simulink library "Contact_Forces_Lib"  (R2024a)
settings: Solver=ode45  StartTime=0.0  StopTime=10.0  RelTol=1e-3  EnableMultiTasking=on
undefined symbols (not defined in the file or in its folder): b_contact, custom_param_1, custom_param_2, Extr_Data_Ring, k_contact, l_cone, length_cylinder, length_tube, mu_kinetic, mu_static, pen_exponent, pen_full_damp_F, rad_s_cone, radius_cylinder, radius_tube, v_thr, X, Y, Z
libraries: nesl_utility x197, sm_lib x115, $bdroot x72, simulink x20, fl_lib x4
(part 10 of 12)

== system Contact_Forces_Lib/3D/Sphere to Tube Force/Forces/Sum ==
  FnxSphF : Inport
  FnySphF : Inport  Port=2
  FnzSphF : Inport  Port=3
  FnxTubB : Inport  Port=4
  FnyTubB : Inport  Port=5
  TnxTubB : Inport  Port=6
  TnyTubB : Inport  Port=7
  FfxSphF : Inport  Port=8
  FfySphF : Inport  Port=9
  FfzSphF : Inport  Port=10
  FfxTubB : Inport  Port=11
  FfyTubB : Inport  Port=12
  FfzTubB : Inport  Port=13
  TzSphF : Inport  Port=14
  TTubB : Inport  Port=15
  Constant : Constant  Value=0
  Mux : Mux  Inputs=3
  Sum{1..6} (6 alike) : Sum
  FxF : Outport  VectorParamsAs1DForOutWhenUnconnected=off
  FyF : Outport  Port=2  VectorParamsAs1DForOutWhenUnconnected=off
  FzF : Outport  Port=3  VectorParamsAs1DForOutWhenUnconnected=off
  TzF : Outport  Port=4  VectorParamsAs1DForOutWhenUnconnected=off
  FxB : Outport  Port=5  VectorParamsAs1DForOutWhenUnconnected=off
  FyB : Outport  Port=6  VectorParamsAs1DForOutWhenUnconnected=off
  FzB : Outport  Port=7  VectorParamsAs1DForOutWhenUnconnected=off
  TB : Outport  Port=8  VectorParamsAs1DForOutWhenUnconnected=off
  wires:
  Sum6/1 -> TB/1
  FfzTubB/1 -> FzB/1
  FfzSphF/1 -> Sum1/2
  FnzSphF/1 -> Sum1/1
  Sum1/1 -> FzF/1
  FnxSphF/1 -> Sum4/1
  FnySphF/1 -> Sum2/1
  FnxTubB/1 -> Sum3/1
  FnyTubB/1 -> Sum5/1
  Sum4/1 -> FxF/1
  Sum2/1 -> FyF/1
  Sum3/1 -> FxB/1
  Sum5/1 -> FyB/1
  FfxSphF/1 -> Sum4/2
  FfySphF/1 -> Sum2/2
  FfxTubB/1 -> Sum3/2
  FfyTubB/1 -> Sum5/2
  TzSphF/1 -> TzF/1
  TTubB/1 -> Sum6/1
  Mux/1 -> Sum6/2
  TnxTubB/1 -> Mux/1
  TnyTubB/1 -> Mux/2
  Constant/1 -> Mux/3

== system Contact_Forces_Lib/3D/Sphere to Tube Force/Sensing/rad_azm_cal ==
  X : Inport
  Y : Inport  Port=2
  Xdot : Inport  Port=3
  Ydot : Inport  Port=4
  Demux : Demux
  If centers are not colocated : If  IfExpression=(u1 > 0)
  Math Function : Math  Operator=square  SignedPower=on
  Math Function1 : Math  Operator=square  SignedPower=on
  Merge : Merge  InitialOutput=0  InputPortOffsets=0
  Sum : Sum  Inputs=|++
  rad_0 : Subsystem
  rad_azm_cal : Subsystem
  rad : Outport  VectorParamsAs1DForOutWhenUnconnected=off
  azm : Outport  Port=2  VectorParamsAs1DForOutWhenUnconnected=off
  radv : Outport  Port=3  VectorParamsAs1DForOutWhenUnconnected=off
  azmv : Outport  Port=4  VectorParamsAs1DForOutWhenUnconnected=off
  wires:
  Sum/1 -> If centers are not colocated/1
  Math Function/1 -> Sum/1
  Math Function1/1 -> Sum/2
  rad_azm_cal/1(F) -> Merge/2
  Y/1 -> rad_azm_cal/2(Y), Math Function1/1
  Ydot/1 -> rad_azm_cal/4(Ydot)
  X/1 -> rad_azm_cal/1(X), Math Function/1
  Xdot/1 -> rad_azm_cal/3(Xdot)
  Demux/3 -> radv/1
  Demux/1 -> rad/1
  Demux/4 -> azmv/1
  rad_0/1(F) -> Merge/1
  Demux/2 -> azm/1
  If centers are not colocated/2 -> rad_0/Action
  If centers are not colocated/1 -> rad_azm_cal/Action
  Merge/1 -> Demux/1

== system Contact_Forces_Lib/3D/Sphere to Tube Force Enabled/Check Active/Check Active Range ==
  azm : Inport
  " Upper Bound" : simulink/Logic and Bit Operations/Compare To Constant  relop=<=  const=active_angle(2)*pi/180  OutDataTypeStr=boolean  ZeroCross=off
  Logical Operator : Logic  AllPortsSameDT=off  OutDataTypeStr=boolean
  Lower Bound : simulink/Logic and Bit Operations/Compare To Constant  relop=>=  const=active_angle(1)*pi/180  OutDataTypeStr=boolean  ZeroCross=off
  En : Outport  VectorParamsAs1DForOutWhenUnconnected=off
  wires:
  Logical Operator/1 -> En/1
  Lower Bound/1 -> Logical Operator/2
  " Upper Bound"/1 -> Logical Operator/1
  azm/1 -> Lower Bound/1, " Upper Bound"/1

== system Contact_Forces_Lib/3D/Sphere to Tube Force Enabled/Check Active/In Tube ==
  z : Inport
  Abs1 : Abs  ZeroCross=off  SaturateOnIntegerOverflow=off
  Activation limit for contact force : Constant  Value=l_tube/2
  Sum : Sum  Inputs=+-
  En : Outport  VectorParamsAs1DForOutWhenUnconnected=off
  wires:
  Sum/1 -> En/1
  Activation limit for contact force/1 -> Sum/1
  z/1 -> Abs1/1
  Abs1/1 -> Sum/2

== system Contact_Forces_Lib/3D/Sphere to Tube Force Enabled/Forces/Calculate Penetration ==
  note: Calculates CirF frame to midpoint of ring wall.
      | Absolute value makes it valid for inside or outside contact.
      | Noting the sign allows us to apply the force correctly
  rad : Inport
  vrad : Inport  Port=2
  Abs : Abs  ZeroCross=off  SaturateOnIntegerOverflow=off
  Constant : Constant  Value=radius_sphere+d_tube/2
  Dead Zone : DeadZone  LowerValue=-inf  UpperValue=0
  Product : Product
  Sign : Signum  ZeroCross=off
  Sum : Sum  Inputs=+-
  Sum1 : Sum  Inputs=+-
  radius ring : Constant  Value=radius_tube
  sign : Outport  VectorParamsAs1DForOutWhenUnconnected=off
  Pen : Outport  Port=2  VectorParamsAs1DForOutWhenUnconnected=off
  Pen Vel : Outport  Port=3  VectorParamsAs1DForOutWhenUnconnected=off
  wires:
  Dead Zone/1 -> Pen/1
  Constant/1 -> Sum/1
  Sum/1 -> Dead Zone/1
  vrad/1 -> Product/2
  Product/1 -> Pen Vel/1
  Sign/1 -> sign/1, Product/1
  Abs/1 -> Sum/2
  rad/1 -> Sum1/2
  Sum1/1 -> Abs/1, Sign/1
  radius ring/1 -> Sum1/1

== system Contact_Forces_Lib/3D/Sphere to Tube Force Enabled/Forces/Ff ==
  note: Sign of Fn indicates if sphere is inside or outside tube
  Fn : Inport
  z : Inport  Port=2
  R : Inport  Port=3
  azm : Inport  Port=4
  vazm : Inport  Port=5
  wzf : Inport  Port=6
  Pen : Inport  Port=7
  rad : Inport  Port=8
  vzf : Inport  Port=9
  wxf : Inport  Port=10
  wyf : Inport  Port=11
  Friction Law : $bdroot/Friction Law  SystemSampleTime=-1  LabelModeActiveChoice=Stick_Slip_C  VariantActivationTime=update diagram  AllowFlexibleInterface=on  Latency=0  AutoFrameSizeCalculation=off
  Relative vel at CP : Subsystem
  Resolve Ff : Subsystem
  Sign : Signum  ZeroCross=off
  FxSphF : Outport  VectorParamsAs1DForOutWhenUnconnected=off
  FySohF : Outport  Port=2  VectorParamsAs1DForOutWhenUnconnected=off
  FzSphF : Outport  Port=3  VectorParamsAs1DForOutWhenUnconnected=off
  FxTubB : Outport  Port=4  VectorParamsAs1DForOutWhenUnconnected=off
  FyTubB : Outport  Port=5  VectorParamsAs1DForOutWhenUnconnected=off
  FzTubB : Outport  Port=6  VectorParamsAs1DForOutWhenUnconnected=off
  TSphF : Outport  Port=7  VectorParamsAs1DForOutWhenUnconnected=off
  TTubB : Outport  Port=8  VectorParamsAs1DForOutWhenUnconnected=off
  Ff : Outport  Port=9  VectorParamsAs1DForOutWhenUnconnected=off
  wires:
  Sign/1 -> Resolve Ff/1(InOut)  "InOut"
  z/1 -> Resolve Ff/6(z)
  Relative vel at CP/1(vRelAbs) -> Friction Law/2  "vRelAbs"
  Relative vel at CP/2(rSphtoCP) -> Resolve Ff/3(rSphtoCP)
  Relative vel at CP/3(rCyltoCP) -> Resolve Ff/4(rCyltoCP)
  azm/1 -> Relative vel at CP/9(azm), Resolve Ff/8(azm)
  wyf/1 -> Relative vel at CP/8(wyf)
  wxf/1 -> Relative vel at CP/7(wxf)
  Resolve Ff/8(TTubB) -> TTubB/1
  Resolve Ff/4(TSphF) -> TSphF/1
  Resolve Ff/6(FyTubB) -> FyTubB/1
  Resolve Ff/5(FxSphB) -> FxTubB/1
  Resolve Ff/2(FySphF) -> FySohF/1
  Resolve Ff/1(FxSphF) -> FxSphF/1
  Friction Law/1 -> Resolve Ff/2(Ff), Ff/1  "Ff Abs"
  wzf/1 -> Relative vel at CP/5(wzf)
  vazm/1 -> Relative vel at CP/4(vazm)
  rad/1 -> Relative vel at CP/2(rad)
  Fn/1 -> Sign/1, Friction Law/1, Relative vel at CP/1(Fn)  "Fn"
  Pen/1 -> Relative vel at CP/3(Pen)
  R/1 -> Resolve Ff/7(R)
  vzf/1 -> Relative vel at CP/6(vzf)
  Relative vel at CP/4(alpha) -> Resolve Ff/5(alpha)
  Resolve Ff/3(FzSphF) -> FzSphF/1
  Resolve Ff/7(FzTubB) -> FzTubB/1

== system Contact_Forces_Lib/3D/Sphere to Tube Force Enabled/Forces/Fn ==
  note: Resolve Normal Force in
      | Sphere F reference frame
  note: Resolve Normal Force in
      | Tube B reference frame
  Fn : Inport
  z : Inport  Port=2
  R : Inport  Port=3
  azm : Inport  Port=4
  Fn in SphF : Subsystem
  Fn in TubB : Subsystem
  Gain : Gain  Gain=-1
  Product : Product
  Product1 : Product
  FxSphF : Outport  VectorParamsAs1DForOutWhenUnconnected=off
  FySphF : Outport  Port=2  VectorParamsAs1DForOutWhenUnconnected=off
  FZSphF : Outport  Port=3  VectorParamsAs1DForOutWhenUnconnected=off
  FxTubB : Outport  Port=4  VectorParamsAs1DForOutWhenUnconnected=off
  FyTubB : Outport  Port=5  VectorParamsAs1DForOutWhenUnconnected=off
  TxTubB : Outport  Port=6  VectorParamsAs1DForOutWhenUnconnected=off
  TyTubB : Outport  Port=7  VectorParamsAs1DForOutWhenUnconnected=off
  wires:
  Fn in SphF/3(FzSphF) -> FZSphF/1
  Fn in SphF/2(FxSphF) -> FxSphF/1
  R/1 -> Fn in SphF/1(R)
  azm/1 -> Fn in TubB/2(azm)
  Fn/1 -> Fn in TubB/1(Fn)
  Fn in TubB/2(FyTubB) -> Fn in SphF/3(FyTubB), FyTubB/1, Gain/1
  Fn in TubB/1(FxTubB) -> Fn in SphF/2(FxTubB), Product/2, FxTubB/1
  Fn in SphF/1(FySphF) -> FySphF/1
  z/1 -> Product1/1, Product/1
  Gain/1 -> Product1/2
  Product/1 -> TyTubB/1
  Product1/1 -> TxTubB/1

== system Contact_Forces_Lib/3D/Sphere to Tube Force Enabled/Forces/Sum ==
  FnxSphF : Inport
  FnySphF : Inport  Port=2
  FnzSphF : Inport  Port=3
  FnxTubB : Inport  Port=4
  FnyTubB : Inport  Port=5
  TnxTubB : Inport  Port=6
  TnyTubB : Inport  Port=7
  FfxSphF : Inport  Port=8
  FfySphF : Inport  Port=9
  FfzSphF : Inport  Port=10
  FfxTubB : Inport  Port=11
  FfyTubB : Inport  Port=12
  FfzTubB : Inport  Port=13
  TzSphF : Inport  Port=14
  TTubB : Inport  Port=15
  Constant : Constant  Value=0
  Mux : Mux  Inputs=3
  Sum{1..6} (6 alike) : Sum
  FxF : Outport  VectorParamsAs1DForOutWhenUnconnected=off
  FyF : Outport  Port=2  VectorParamsAs1DForOutWhenUnconnected=off
  FzF : Outport  Port=3  VectorParamsAs1DForOutWhenUnconnected=off
  TzF : Outport  Port=4  VectorParamsAs1DForOutWhenUnconnected=off
  FxB : Outport  Port=5  VectorParamsAs1DForOutWhenUnconnected=off
  FyB : Outport  Port=6  VectorParamsAs1DForOutWhenUnconnected=off
  FzB : Outport  Port=7  VectorParamsAs1DForOutWhenUnconnected=off
  TB : Outport  Port=8  VectorParamsAs1DForOutWhenUnconnected=off
  wires:
  Sum6/1 -> TB/1
  FfzTubB/1 -> FzB/1
  FfzSphF/1 -> Sum1/2
  FnzSphF/1 -> Sum1/1
  Sum1/1 -> FzF/1
  FnxSphF/1 -> Sum4/1
  FnySphF/1 -> Sum2/1
  FnxTubB/1 -> Sum3/1
  FnyTubB/1 -> Sum5/1
  Sum4/1 -> FxF/1
  Sum2/1 -> FyF/1
  Sum3/1 -> FxB/1
  Sum5/1 -> FyB/1
  FfxSphF/1 -> Sum4/2
  FfySphF/1 -> Sum2/2
  FfxTubB/1 -> Sum3/2
  FfyTubB/1 -> Sum5/2
  TzSphF/1 -> TzF/1
  TTubB/1 -> Sum6/1
  Mux/1 -> Sum6/2
  TnxTubB/1 -> Mux/1
  TnyTubB/1 -> Mux/2
  Constant/1 -> Mux/3

== system Contact_Forces_Lib/3D/Sphere to Tube Force Enabled/Sensing/In or Out ==
  rad : Inport
  Constant : Constant  Value=radius_tube
  Constant1 : Constant  Value=-d_tube/2
  Constant2 : Constant  Value=radius_tube
  Product : Product
  Product1 : Product
  Sign : Signum  ZeroCross=off
  Subtract : Sum  Inputs=+-
  Sum : Sum
  factor : Outport  VectorParamsAs1DForOutWhenUnconnected=off
  wires:
  Constant/1 -> Subtract/1
  Sign/1 -> Product/1, Product1/1
  Subtract/1 -> Sign/1
  rad/1 -> Subtract/2
  Constant1/1 -> Product/2
  Product/1 -> Sum/1
  Sum/1 -> Product1/2
  Product1/1 -> factor/1
  Constant2/1 -> Sum/2

== system Contact_Forces_Lib/3D/Sphere to Tube Force Enabled/Sensing/rad_azm_cal ==
  X : Inport
  Y : Inport  Port=2
  Xdot : Inport  Port=3
  Ydot : Inport  Port=4
  Demux : Demux
  If centers are not colocated : If  IfExpression=(u1 > 0)
  Math Function : Math  Operator=square  SignedPower=on
  Math Function1 : Math  Operator=square  SignedPower=on
  Merge : Merge  InitialOutput=0  InputPortOffsets=0
  Sum : Sum  Inputs=|++
  rad_0 : Subsystem
  rad_azm_cal : Subsystem
  rad : Outport  VectorParamsAs1DForOutWhenUnconnected=off
  azm : Outport  Port=2  VectorParamsAs1DForOutWhenUnconnected=off
  radv : Outport  Port=3  VectorParamsAs1DForOutWhenUnconnected=off
  azmv : Outport  Port=4  VectorParamsAs1DForOutWhenUnconnected=off
  wires:
  Sum/1 -> If centers are not colocated/1
  Math Function/1 -> Sum/1
  Math Function1/1 -> Sum/2
  rad_azm_cal/1(F) -> Merge/2
  Y/1 -> rad_azm_cal/2(Y), Math Function1/1
  Ydot/1 -> rad_azm_cal/4(Ydot)
  X/1 -> rad_azm_cal/1(X), Math Function/1
  Xdot/1 -> rad_azm_cal/3(Xdot)
  Demux/3 -> radv/1
  Demux/1 -> rad/1
  Demux/4 -> azmv/1
  rad_0/1(F) -> Merge/1
  Demux/2 -> azm/1
  If centers are not colocated/2 -> rad_0/Action
  If centers are not colocated/1 -> rad_azm_cal/Action
  Merge/1 -> Demux/1

== system Contact_Forces_Lib/Friction Utilities/Utilities/Product/FcConst ==
  PS Product : fl_lib/Physical Signals/Functions/PS Product
  PS Terminator : fl_lib/Physical Signals/Sinks/PS Terminator
  Fc : PMIOPort  Side=Right
  v : PMIOPort  Port=2  Side=Right
  connections:
  PS Product/LConn1 -- v/RConn1
  PS Product/LConn2 -- Fc/RConn1
  PS Terminator/LConn1 -- PS Product/RConn1

== system Contact_Forces_Lib/Friction Utilities/Utilities/Product/FcVect ==
  PS Terminator : fl_lib/Physical Signals/Sinks/PS Terminator
  PS Terminator1 : fl_lib/Physical Signals/Sinks/PS Terminator
  Fc : PMIOPort  Side=Right
  v : PMIOPort  Port=2  Side=Right
  connections:
  PS Terminator1/LConn1 -- Fc/RConn1
  PS Terminator/LConn1 -- v/RConn1

== system Contact_Forces_Lib/2D/Circle to Circle Force/Ff/Resolve Ff/Ff in CirB ==
  Ff : Inport
  azm : Inport  Port=2
  Divide1 : Product  Inputs=**
  Divide2 : Product  Inputs=**
  Gain3 : Gain  Gain=-1
  cos : Trigonometry
  deg2rad : Gain  Gain=pi/180
  sin : Trigonometry  Operator=cos
  FxCirB : Outport  VectorParamsAs1DForOutWhenUnconnected=off
  FyCirB : Outport  Port=2  VectorParamsAs1DForOutWhenUnconnected=off
  wires:
  Gain3/1 -> Divide1/2
  Ff/1 -> Divide1/1, Divide2/1
  Divide1/1 -> FxCirB/1
  deg2rad/1 -> cos/1, sin/1
  sin/1 -> Divide2/2
  cos/1 -> Gain3/1
  Divide2/1 -> FyCirB/1  "Fy Cir"
  azm/1 -> deg2rad/1

== system Contact_Forces_Lib/2D/Circle to Circle Force/Ff/Resolve Ff/Ff in CirF ==
  R : Inport
  FxCirB : Inport  Port=2
  FyCirB : Inport  Port=3
  Demux : Demux  Outputs=2
  Divide3 : Product  Inputs=**  Multiplication=Matrix(*)
  Gain1 : Gain  Gain=-1
  Mux1 : Mux  Inputs=2
  FyCirF : Outport  VectorParamsAs1DForOutWhenUnconnected=off
  FxCirF : Outport  Port=2  VectorParamsAs1DForOutWhenUnconnected=off
  wires:
  FxCirB/1 -> Mux1/2
  FyCirB/1 -> Mux1/1
  Demux/2 -> FxCirF/1
  Demux/1 -> FyCirF/1
  Gain1/1 -> Demux/1
  Mux1/1 -> Divide3/2
  Divide3/1 -> Gain1/1
  R/1 -> Divide3/1

== system Contact_Forces_Lib/2D/Circle to Circle Force/Ff/Resolve Ff/Tz ==
  rCirFtoCP : Inport
  rCirBtoCP : Inport  Port=2
  Ff : Inport  Port=3
  Divide4 : Product  Inputs=**
  Divide5 : Product  Inputs=**
  Gain2 : Gain
  TzB : Outport  VectorParamsAs1DForOutWhenUnconnected=off
  TzF : Outport  Port=2  VectorParamsAs1DForOutWhenUnconnected=off
  wires:
  Ff/1 -> Divide4/1, Gain2/1
  Gain2/1 -> Divide5/1
  Divide4/1 -> TzF/1
  rCirFtoCP/1 -> Divide4/2
  Divide5/1 -> TzB/1
  rCirBtoCP/1 -> Divide5/2

== system Contact_Forces_Lib/2D/Circle to Circle Force Enabled/Ff/Resolve Ff/Ff in CirB ==
  Ff : Inport
  azm : Inport  Port=2
  Divide1 : Product  Inputs=**
  Divide2 : Product  Inputs=**
  Gain3 : Gain  Gain=-1
  cos : Trigonometry
  deg2rad : Gain  Gain=pi/180
  sin : Trigonometry  Operator=cos
  FxCirB : Outport  VectorParamsAs1DForOutWhenUnconnected=off
  FyCirB : Outport  Port=2  VectorParamsAs1DForOutWhenUnconnected=off
  wires:
  azm/1 -> deg2rad/1
  Divide2/1 -> FyCirB/1  "Fy Cir"
  cos/1 -> Gain3/1
  sin/1 -> Divide2/2
  deg2rad/1 -> sin/1, cos/1
  Divide1/1 -> FxCirB/1
  Ff/1 -> Divide2/1, Divide1/1
  Gain3/1 -> Divide1/2

== system Contact_Forces_Lib/2D/Circle to Circle Force Enabled/Ff/Resolve Ff/Ff in CirF ==
  R : Inport
  FxCirB : Inport  Port=2
  FyCirB : Inport  Port=3
  Demux : Demux  Outputs=2
  Divide3 : Product  Inputs=**  Multiplication=Matrix(*)
  Gain1 : Gain  Gain=-1
  Mux1 : Mux  Inputs=2
  FyCirF : Outport  VectorParamsAs1DForOutWhenUnconnected=off
  FxCirF : Outport  Port=2  VectorParamsAs1DForOutWhenUnconnected=off
  wires:
  R/1 -> Divide3/1
  Divide3/1 -> Gain1/1
  Mux1/1 -> Divide3/2
  Gain1/1 -> Demux/1
  Demux/1 -> FyCirF/1
  Demux/2 -> FxCirF/1
  FyCirB/1 -> Mux1/1
  FxCirB/1 -> Mux1/2

== system Contact_Forces_Lib/2D/Circle to Circle Force Enabled/Ff/Resolve Ff/Tz ==
  rCirFtoCP : Inport
  rCirBtoCP : Inport  Port=2
  Ff : Inport  Port=3
  Divide4 : Product  Inputs=**
  Divide5 : Product  Inputs=**
  Gain2 : Gain
  TzB : Outport  VectorParamsAs1DForOutWhenUnconnected=off
  TzF : Outport  Port=2  VectorParamsAs1DForOutWhenUnconnected=off
  wires:
  rCirBtoCP/1 -> Divide5/2
  Divide5/1 -> TzB/1
  rCirFtoCP/1 -> Divide4/2
  Divide4/1 -> TzF/1
  Gain2/1 -> Divide5/1
  Ff/1 -> Gain2/1, Divide4/1

== system Contact_Forces_Lib/2D/Circle to Finite Line Force/Forces/Resolve Forces/FnCir ==
  note: Calculate circle Normal Force in circle reference frame
  Unit Vector : Inport
  Fn : Inport  Port=2
  Demux1 : Demux  Outputs=2
  Divide1 : Product  Inputs=**
  FxCir : Outport  VectorParamsAs1DForOutWhenUnconnected=off
  FyCir : Outport  Port=2  VectorParamsAs1DForOutWhenUnconnected=off
  wires:
  Unit Vector/1 -> Divide1/2
  Divide1/1 -> Demux1/1
  Fn/1 -> Divide1/1
  Demux1/2 -> FyCir/1  "Fy Cir"
  Demux1/1 -> FxCir/1  "Fx Cir"

== system Contact_Forces_Lib/2D/Circle to Finite Line Force/Forces/Resolve Forces/FnLin ==
  note: Normal Force is calculated in line reference frame,
      | and acts along x-axis only.
  Fn : Inport
  Constant : Constant  Value=0
  Constant1 : Constant  Value=0
  Sum : Sum
  FxLin : Outport  VectorParamsAs1DForOutWhenUnconnected=off
  FyLin : Outport  Port=2  VectorParamsAs1DForOutWhenUnconnected=off
  wires:
  Constant1/1 -> Sum/1
  Sum/1 -> FxLin/1
  Fn/1 -> Sum/2  "Fx Lin"
  Constant/1 -> FyLin/1  "Fy Lin"

== system Contact_Forces_Lib/2D/Circle to Finite Line Force/Forces/Resolve Forces/Friction ==
  Unit Vector : Inport
  Fn : Inport  Port=2
  X Sep : Inport  Port=3
  vLin : Inport  Port=4
  wz : Inport  Port=5
  Components : Gain  Gain=[1 -1]
  Demux : Demux  Outputs=2
  Friction Law : $bdroot/Friction Law  SystemSampleTime=-1  LabelModeActiveChoice=None  VariantActivationTime=update diagram  AllowFlexibleInterface=on  Latency=0  AutoFrameSizeCalculation=off
  Line Ref h : Gain  Gain=line_depth
  Product1 : Product
  Product2 : Product
  Product3 : Product
  Radius : Gain  Gain=-circle_rad
  Sign : Signum
  Sum : Sum  Inputs=-+
  VCirPt : Subsystem
  FxCir : Outport  VectorParamsAs1DForOutWhenUnconnected=off
  FyCir : Outport  Port=2  VectorParamsAs1DForOutWhenUnconnected=off
  FyLin : Outport  Port=3  VectorParamsAs1DForOutWhenUnconnected=off
  TzLin : Outport  Port=4  VectorParamsAs1DForOutWhenUnconnected=off
  TzCir : Outport  Port=5  VectorParamsAs1DForOutWhenUnconnected=off
  Ff : Outport  Port=6  VectorParamsAs1DForOutWhenUnconnected=off
  wires:
  Sign/1 -> Product3/2, Product1/2
  X Sep/1 -> VCirPt/2(X sep), Sign/1
  Product2/1 -> Demux/1
  Radius/1 -> TzCir/1
  Line Ref h/1 -> TzLin/1
  Fn/1 -> Friction Law/1
  Sum/1 -> Friction Law/2
  Unit Vector/1 -> Components/1
  wz/1 -> VCirPt/1(wz)
  Demux/2 -> FxCir/1  "FxCir"
  VCirPt/1(vCir) -> Sum/2
  vLin/1 -> Sum/1
  Demux/1 -> FyCir/1  "FyCir"
  Friction Law/1 -> Product1/1, Radius/1, Ff/1, Product2/2, Line Ref h/1  "Ff"
  Product1/1 -> FyLin/1
  Components/1 -> Product3/1
  Product3/1 -> Product2/1

== system Contact_Forces_Lib/2D/Circle to Finite Line Force Enabled/Forces/Resolve Forces/FnCir ==
  note: Calculate circle Normal Force in circle reference frame
  Unit Vector : Inport
  Fn : Inport  Port=2
  Demux1 : Demux  Outputs=2
  Divide1 : Product  Inputs=**
  FxCir : Outport  VectorParamsAs1DForOutWhenUnconnected=off
  FyCir : Outport  Port=2  VectorParamsAs1DForOutWhenUnconnected=off
  wires:
  Demux1/1 -> FxCir/1  "Fx Cir"
  Demux1/2 -> FyCir/1  "Fy Cir"
  Fn/1 -> Divide1/1
  Divide1/1 -> Demux1/1
  Unit Vector/1 -> Divide1/2

== system Contact_Forces_Lib/2D/Circle to Finite Line Force Enabled/Forces/Resolve Forces/FnLin ==
  note: Normal Force is calculated in line reference frame,
      | and acts along x-axis only.
  Fn : Inport
  Constant : Constant  Value=0
  Constant1 : Constant  Value=0
  Sum : Sum
  FxLin : Outport  VectorParamsAs1DForOutWhenUnconnected=off
  FyLin : Outport  Port=2  VectorParamsAs1DForOutWhenUnconnected=off
  wires:
  Constant/1 -> FyLin/1  "Fy Lin"
  Fn/1 -> Sum/2  "Fx Lin"
  Sum/1 -> FxLin/1
  Constant1/1 -> Sum/1

== system Contact_Forces_Lib/2D/Circle to Finite Line Force Enabled/Forces/Resolve Forces/Friction ==
  Unit Vector : Inport
  Fn : Inport  Port=2
  X Sep : Inport  Port=3
  vLin : Inport  Port=4
  wz : Inport  Port=5
  Components : Gain  Gain=[1 -1]
  Demux : Demux  Outputs=2
  Friction Law : $bdroot/Friction Law  SystemSampleTime=-1  LabelModeActiveChoice=None  VariantActivationTime=update diagram  AllowFlexibleInterface=on  Latency=0  AutoFrameSizeCalculation=off
  Line Ref h : Gain  Gain=line_depth
  Product1 : Product
  Product2 : Product
  Product3 : Product
  Radius : Gain  Gain=-circle_rad
  Sign : Signum
  Sum : Sum  Inputs=-+
  VCirPt : Subsystem
  FxCir : Outport  VectorParamsAs1DForOutWhenUnconnected=off
  FyCir : Outport  Port=2  VectorParamsAs1DForOutWhenUnconnected=off
  FyLin : Outport  Port=3  VectorParamsAs1DForOutWhenUnconnected=off
  TzLin : Outport  Port=4  VectorParamsAs1DForOutWhenUnconnected=off
  TzCir : Outport  Port=5  VectorParamsAs1DForOutWhenUnconnected=off
  Ff : Outport  Port=6  VectorParamsAs1DForOutWhenUnconnected=off
  wires:
  Product3/1 -> Product2/1
  Components/1 -> Product3/1
  Product1/1 -> FyLin/1
  Friction Law/1 -> Line Ref h/1, Product2/2, Ff/1, Radius/1, Product1/1  "Ff"
  Demux/1 -> FyCir/1  "FyCir"
  vLin/1 -> Sum/1
  VCirPt/1(vCir) -> Sum/2
  Demux/2 -> FxCir/1  "FxCir"
  wz/1 -> VCirPt/1(wz)
  Unit Vector/1 -> Components/1
  Sum/1 -> Friction Law/2
  Fn/1 -> Friction Law/1
  Line Ref h/1 -> TzLin/1
  Radius/1 -> TzCir/1
  Product2/1 -> Demux/1
  X Sep/1 -> Sign/1, VCirPt/2(X sep)
  Sign/1 -> Product1/2, Product3/2

== system Contact_Forces_Lib/2D/Circle to Ring Force/Forces/Ff/Calculate vRel at CP  ==
  InOut : Inport
  rad : Inport  Port=2
  Pen : Inport  Port=3
  vazm : Inport  Port=4
  wzf : Inport  Port=5
  Follower Radius : Constant  Value=radius_circle
  Midpt Pen : Gain  Gain=0.5
  Product1 : Product
  Product2 : Product
  Product3 : Product
  Sum{,1..2,4} (4 alike) : Sum  Inputs=+-
  vRelCP : Outport  VectorParamsAs1DForOutWhenUnconnected=off
  rCirFtoCP : Outport  Port=2  VectorParamsAs1DForOutWhenUnconnected=off
  rRinBtoCP : Outport  Port=3  VectorParamsAs1DForOutWhenUnconnected=off
  wires:
  InOut/1 -> Product1/2  "InOut"
  Sum2/1 -> vRelCP/1
  Pen/1 -> Midpt Pen/1
  Sum/1 -> rRinBtoCP/1, Product2/2  "rRinBtoCP"
  rad/1 -> Sum/1
  Product2/1 -> Sum2/1  "vRelTra"
  Product3/1 -> Sum2/2  "vRelRot"
  Follower Radius/1 -> Sum1/1
  wzf/1 -> Sum4/1
  vazm/1 -> Product2/1, Sum4/2
  Midpt Pen/1 -> Sum1/2
  Sum4/1 -> Product3/1
  Product1/1 -> Sum/2, Product3/2  "rCirFtoCP sign"
  Sum1/1 -> rCirFtoCP/1, Product1/1  "rCirFtoCP"

== system Contact_Forces_Lib/2D/Circle to Ring Force/Forces/Ff/Resolve Ff ==
  note: Resolve Friction Force in
      | Circle B reference frame
      | Sign of Fn indicates
      | inside or outside ring.
  note: Resolve Friction Force in
      | Circle F reference frame
  Fn : Inport
  Ff : Inport  Port=2
  R : Inport  Port=3
  azm : Inport  Port=4
  rCirFtoCP : Inport  Port=5
  rRinBtoCP : Inport  Port=6
  Ff in CirB : Subsystem
  Ff in CirF : Subsystem
  Product : Product
  Sign : Signum  ZeroCross=off
  Tz : Subsystem
  FxCirF : Outport  VectorParamsAs1DForOutWhenUnconnected=off
  FyCirF : Outport  Port=2  VectorParamsAs1DForOutWhenUnconnected=off
  TzCirF : Outport  Port=3  VectorParamsAs1DForOutWhenUnconnected=off
  FxRinB : Outport  Port=4  VectorParamsAs1DForOutWhenUnconnected=off
  FyRinB : Outport  Port=5  VectorParamsAs1DForOutWhenUnconnected=off
  TzRinB : Outport  Port=6  VectorParamsAs1DForOutWhenUnconnected=off
  wires:
  Product/1 -> Ff in CirB/1(Ff)
  Sign/1 -> Product/2
  Fn/1 -> Sign/1
  Ff in CirF/1(FyCirF) -> FyCirF/1
  Ff in CirB/1(FxRinB) -> FxRinB/1, Ff in CirF/2(FxRinB)
  Ff in CirB/2(FyRinB) -> FyRinB/1, Ff in CirF/3(FyRinB)
  Ff in CirF/2(FxCirF) -> FxCirF/1
  Ff/1 -> Product/1, Tz/3(Ff)
  Tz/1(TzRinB) -> TzRinB/1
  Tz/2(TzCirF) -> TzCirF/1
  azm/1 -> Ff in CirB/2(azm)
  R/1 -> Ff in CirF/1(R)
  rCirFtoCP/1 -> Tz/1(rCirFtoCP)
  rRinBtoCP/1 -> Tz/2(rRinBtoCP)

== system Contact_Forces_Lib/2D/Circle to Ring Force/Forces/Fn/Fn in CirB ==
  Fn : Inport
  azm : Inport  Port=2
  Divide1 : Product  Inputs=**
  Divide2 : Product  Inputs=**
  Gain2 : Gain  Gain=-1
  cos : Trigonometry  Operator=cos
  deg2rad : Gain  Gain=pi/180
  sin : Trigonometry
  FxCirB : Outport  VectorParamsAs1DForOutWhenUnconnected=off
  FyCirB : Outport  Port=2  VectorParamsAs1DForOutWhenUnconnected=off
  wires:
  Gain2/1 -> Divide1/1, Divide2/1
  deg2rad/1 -> cos/1, sin/1
  sin/1 -> Divide2/2
  cos/1 -> Divide1/2
  Divide1/1 -> FxCirB/1
  Divide2/1 -> FyCirB/1
  Fn/1 -> Gain2/1
  azm/1 -> deg2rad/1

== system Contact_Forces_Lib/2D/Circle to Ring Force/Forces/Fn/Fn in CirF ==
  R : Inport
  FxCirB : Inport  Port=2
  FyCirB : Inport  Port=3
  Demux : Demux  Outputs=2
  Divide3 : Product  Inputs=**  Multiplication=Matrix(*)
  Gain : Gain  Gain=-1
  Mux1 : Mux  Inputs=2
  FyCirF : Outport  VectorParamsAs1DForOutWhenUnconnected=off
  FxCirF : Outport  Port=2  VectorParamsAs1DForOutWhenUnconnected=off
  wires:
  Demux/2 -> FxCirF/1
  Demux/1 -> FyCirF/1
  Gain/1 -> Demux/1
  Mux1/1 -> Divide3/2
  Divide3/1 -> Gain/1
  R/1 -> Divide3/1
  FyCirB/1 -> Mux1/1
  FxCirB/1 -> Mux1/2

== system Contact_Forces_Lib/2D/Composite Forces/Box to Belt Force/Belt Ends/Sensing C5 ==
  S : Inport
  Bus Selector : BusSelector  OutputSignals=Normal Force
  Fn : Outport  VectorParamsAs1DForOutWhenUnconnected=off
  wires:
  S/1 -> Bus Selector/1
  Bus Selector/1 -> Fn/1  "<Normal Force>"

== system Contact_Forces_Lib/2D/Composite Forces/Box to Belt Force/Belt Ends/Sensing C6 ==
  S : Inport
  Bus Selector : BusSelector  OutputSignals=Normal Force
  Fn : Outport  VectorParamsAs1DForOutWhenUnconnected=off
  wires:
  Bus Selector/1 -> Fn/1  "<Normal Force>"
  S/1 -> Bus Selector/1

== system Contact_Forces_Lib/2D/Composite Forces/Box to Belt Force/Belt Ends/Sensing C7 ==
  S : Inport
  Bus Selector : BusSelector  OutputSignals=Normal Force
  Fn : Outport  VectorParamsAs1DForOutWhenUnconnected=off
  wires:
  Bus Selector/1 -> Fn/1  "<Normal Force>"
  S/1 -> Bus Selector/1

== system Contact_Forces_Lib/2D/Composite Forces/Box to Belt Force/Belt Ends/Sensing C8 ==
  S : Inport
  Bus Selector : BusSelector  OutputSignals=Normal Force
  Fn : Outport  VectorParamsAs1DForOutWhenUnconnected=off
  wires:
  S/1 -> Bus Selector/1
  Bus Selector/1 -> Fn/1  "<Normal Force>"

== system Contact_Forces_Lib/2D/Composite Forces/Box to Belt Force/Belt Faces/Sensing C1 ==
  S : Inport
  Bus Selector : BusSelector  OutputSignals=Normal Force
  Fn : Outport  VectorParamsAs1DForOutWhenUnconnected=off
  wires:
  Bus Selector/1 -> Fn/1  "<Normal Force>"
  S/1 -> Bus Selector/1

== system Contact_Forces_Lib/2D/Composite Forces/Box to Belt Force/Belt Faces/Sensing C2 ==
  S : Inport
  Bus Selector : BusSelector  OutputSignals=Normal Force
  Fn : Outport  VectorParamsAs1DForOutWhenUnconnected=off
  wires:
  S/1 -> Bus Selector/1
  Bus Selector/1 -> Fn/1  "<Normal Force>"

== system Contact_Forces_Lib/2D/Composite Forces/Box to Belt Force/Belt Faces/Sensing C3 ==
  S : Inport
  Bus Selector : BusSelector  OutputSignals=Normal Force
  Fn : Outport  VectorParamsAs1DForOutWhenUnconnected=off
  wires:
  S/1 -> Bus Selector/1
  Bus Selector/1 -> Fn/1  "<Normal Force>"

== system Contact_Forces_Lib/2D/Composite Forces/Box to Belt Force/Belt Faces/Sensing C4 ==
  S : Inport
  Bus Selector : BusSelector  OutputSignals=Normal Force
  Fn : Outport  VectorParamsAs1DForOutWhenUnconnected=off
  wires:
  Bus Selector/1 -> Fn/1  "<Normal Force>"
  S/1 -> Bus Selector/1

== system Contact_Forces_Lib/2D/Composite Forces/Box to Box Force/BoxB Corners/Forces ==
  1AC : Inport
  1BD : Inport  Port=2
  2AC : Inport  Port=3
  2BD : Inport  Port=4
  3AC : Inport  Port=5
  3BD : Inport  Port=6
  4AC : Inport  Port=7
  4BD : Inport  Port=8
  Bus Creator : BusCreator  Inputs=8
  Bus Selector{1..8} (8 alike) : BusSelector  OutputSignals=FLin.Fx  OutputAsBus=on
  tag scope: FrcBC=scoped
  wires:
  Bus Creator/1 -> [FrcBC]
  Bus Selector7/1 -> Bus Creator/8  "BC4BD"
  4BD/1 -> Bus Selector7/1
  Bus Selector8/1 -> Bus Creator/7  "BC4AC"
  4AC/1 -> Bus Selector8/1
  Bus Selector5/1 -> Bus Creator/6  "BC3BD"
  3BD/1 -> Bus Selector5/1
  Bus Selector6/1 -> Bus Creator/5  "BC3AC"
  3AC/1 -> Bus Selector6/1
  Bus Selector3/1 -> Bus Creator/4  "BC2BD"
  2BD/1 -> Bus Selector3/1
  Bus Selector4/1 -> Bus Creator/3  "BC2AC"
  2AC/1 -> Bus Selector4/1
  Bus Selector1/1 -> Bus Creator/2  "BC1BD"
  1BD/1 -> Bus Selector1/1
  Bus Selector2/1 -> Bus Creator/1  "BC1AC"
  1AC/1 -> Bus Selector2/1

== system Contact_Forces_Lib/2D/Composite Forces/Box to Box Force/BoxF Corners/Forces ==
  1AC : Inport
  1BD : Inport  Port=2
  2AC : Inport  Port=3
  2BD : Inport  Port=4
  3AC : Inport  Port=5
  3BD : Inport  Port=6
  4AC : Inport  Port=7
  4BD : Inport  Port=8
  Bus Creator : BusCreator  Inputs=8
  Bus Selector{1..8} (8 alike) : BusSelector  OutputSignals=FLin.Fx  OutputAsBus=on
  tag scope: FrcFC=scoped
  wires:
  Bus Creator/1 -> [FrcFC]
  Bus Selector7/1 -> Bus Creator/8  "FC4BD"
  4BD/1 -> Bus Selector7/1
  Bus Selector8/1 -> Bus Creator/7  "FC4AC"
  4AC/1 -> Bus Selector8/1
  Bus Selector5/1 -> Bus Creator/6  "FC3BD"
  3BD/1 -> Bus Selector5/1
  Bus Selector6/1 -> Bus Creator/5  "FC3AC"
  3AC/1 -> Bus Selector6/1
  Bus Selector3/1 -> Bus Creator/4  "FC2BD"
  2BD/1 -> Bus Selector3/1
  Bus Selector4/1 -> Bus Creator/3  "FC2AC"
  2AC/1 -> Bus Selector4/1
  Bus Selector1/1 -> Bus Creator/2  "FC1BD"
  1BD/1 -> Bus Selector1/1
  Bus Selector2/1 -> Bus Creator/1  "FC1AC"
  1AC/1 -> Bus Selector2/1

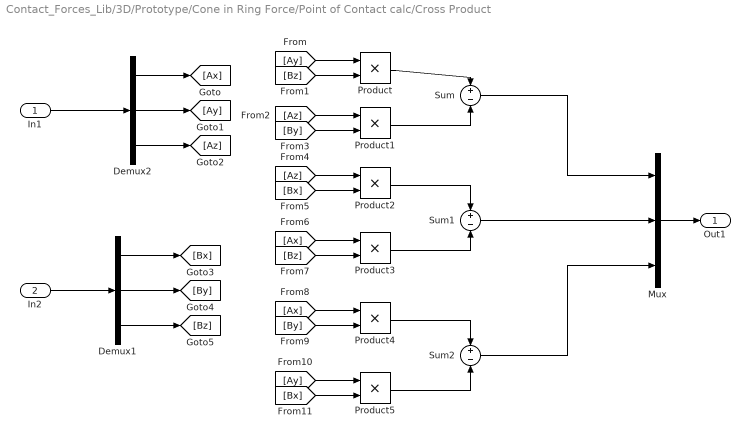
== system Contact_Forces_Lib/3D/Prototype/Cone in Ring Force/Point of Contact calc/Cross Product ==
  In1 : Inport
  In2 : Inport  Port=2
  Demux1 : Demux  Outputs=3
  Demux2 : Demux  Outputs=3
  Mux : Mux  Inputs=3
  Product{,1..5} (6 alike) : Product
  Sum : Sum  Inputs=+|-
  Sum1 : Sum  Inputs=+|-
  Sum2 : Sum  Inputs=+|-
  Out1 : Outport  VectorParamsAs1DForOutWhenUnconnected=off
  wires:
  [Bx] -> Product5/2
  [Ay] -> Product5/1
  [By] -> Product4/2
  [Ax] -> Product4/1
  [Bz] -> Product3/2
  [Ax] -> Product3/1
  [Bx] -> Product2/2
  [Az] -> Product2/1
  [By] -> Product1/2
  [Az] -> Product1/1
  [Bz] -> Product/2
  [Ay] -> Product/1
  Demux1/3 -> [Bz]
  Demux1/2 -> [By]
  Demux1/1 -> [Bx]
  Demux2/3 -> [Az]
  Demux2/2 -> [Ay]
  Demux2/1 -> [Ax]
  In1/1 -> Demux2/1
  Sum2/1 -> Mux/3
  Sum/1 -> Mux/1
  Sum1/1 -> Mux/2
  Product5/1 -> Sum2/2
  Product4/1 -> Sum2/1
  Product3/1 -> Sum1/2
  Product2/1 -> Sum1/1
  Product/1 -> Sum/1
  Product1/1 -> Sum/2
  Mux/1 -> Out1/1
  In2/1 -> Demux1/1

== system Contact_Forces_Lib/3D/Prototype/Cone in Ring Force/Point of Contact calc/Force Calc ==
  x : Inport
  y : Inport  Port=2
  r : Inport  Port=3
  z : Inport  Port=4
  th : Inport  Port=5
  Computing Force from nonzero penetration points : Subsystem  Commented=on
  Constant2 : Constant  Value=r_tube
  Dead Zone : DeadZone  LowerValue=-inf  UpperValue=0  ZeroCross=off
  MAX_ML : Subsystem  Commented=on
  MAX_SL : Subsystem
  Math Function : Math  Operator=square  SignedPower=on
  Math Function1 : Math  Operator=square  SignedPower=on
  Reciprocal Sqrt : Sqrt
  Sum : Sum  Inputs=|++
  Sum1 : Sum  Inputs=|+-
  Fx : Outport  VectorParamsAs1DForOutWhenUnconnected=off
  Fy : Outport  Port=2  VectorParamsAs1DForOutWhenUnconnected=off
  Fz : Outport  Port=3  VectorParamsAs1DForOutWhenUnconnected=off
  pc : Outport  Port=4  VectorParamsAs1DForOutWhenUnconnected=off
  wires:
  x/1 -> MAX_SL/2(X), Math Function/1
  Sum/1 -> Reciprocal Sqrt/1
  Reciprocal Sqrt/1 -> Sum1/1
  Constant2/1 -> Sum1/2
  Sum1/1 -> Dead Zone/1
  Math Function1/1 -> Sum/1
  Math Function/1 -> Sum/2
  y/1 -> Math Function1/1, MAX_SL/1(Y)
  MAX_SL/1(Fx) -> Fx/1
  MAX_SL/2(Fy) -> Fy/1
  Dead Zone/1 -> MAX_SL/3(Pen)
  MAX_SL/3(Fz) -> Fz/1
  MAX_SL/4(pc) -> pc/1
  r/1 -> MAX_SL/4(r)
  th/1 -> MAX_SL/5(th)
  z/1 -> MAX_SL/6(z)

== system Contact_Forces_Lib/3D/Prototype/Cone in Ring Force/Point of Contact calc/r calc ==
  note: r(z) = (z+l_cyl/2)(rl-rs)/lc +rl
  z : Inport
  Constant4 : Constant  Value=(rl + (l_cyl*(rl - rs))/(2*lc))
  Gain1 : Gain  Gain=(rl - rs)/lc
  Sum1 : Sum  Inputs=|++
  r : Outport  VectorParamsAs1DForOutWhenUnconnected=off
  wires:
  Constant4/1 -> Sum1/2
  Gain1/1 -> Sum1/1
  z/1 -> Gain1/1
  Sum1/1 -> r/1

== system Contact_Forces_Lib/3D/Prototype/Cone in Ring Force/Point of Contact calc/x calc ==
  r11 : Inport
  r12 : Inport  Port=2
  r13 : Inport  Port=3
  xc : Inport  Port=4
  th : Inport  Port=5
  z : Inport  Port=6
  r : Inport  Port=7
  Product{,1..4} (5 alike) : Product
  Sum : Sum  Inputs=|++++
  Trigonometric Function : Trigonometry  Operator=cos
  Trigonometric Function1 : Trigonometry
  x : Outport  VectorParamsAs1DForOutWhenUnconnected=off
  wires:
  th/1 -> Trigonometric Function1/1, Trigonometric Function/1
  Sum/1 -> x/1
  Product/1 -> Product3/1
  Product4/1 -> Sum/3
  Trigonometric Function/1 -> Product/2
  Trigonometric Function1/1 -> Product1/2
  Product3/1 -> Sum/2
  Product1/1 -> Product4/2
  r11/1 -> Product/1
  r12/1 -> Product1/1
  xc/1 -> Sum/1
  r13/1 -> Product2/1
  z/1 -> Product2/2
  Product2/1 -> Sum/4
  r/1 -> Product3/2, Product4/1

== system Contact_Forces_Lib/3D/Prototype/Cone in Ring Force/Point of Contact calc/y calc ==
  r21 : Inport
  r22 : Inport  Port=2
  r23 : Inport  Port=3
  yc : Inport  Port=4
  th : Inport  Port=5
  z : Inport  Port=6
  r : Inport  Port=7
  Product{,1..4} (5 alike) : Product
  Sum : Sum  Inputs=|++++
  Trigonometric Function : Trigonometry  Operator=cos
  Trigonometric Function1 : Trigonometry
  y : Outport  VectorParamsAs1DForOutWhenUnconnected=off
  wires:
  Product2/1 -> Sum/4
  z/1 -> Product2/2
  r23/1 -> Product2/1
  yc/1 -> Sum/1
  r22/1 -> Product1/1
  r21/1 -> Product/1
  Product1/1 -> Product4/2
  Product3/1 -> Sum/2
  Trigonometric Function1/1 -> Product1/2
  Trigonometric Function/1 -> Product/2
  Product4/1 -> Sum/3
  Product/1 -> Product3/1
  Sum/1 -> y/1
  th/1 -> Trigonometric Function1/1, Trigonometric Function/1
  r/1 -> Product3/2, Product4/1

== system Contact_Forces_Lib/3D/Prototype/Cone in Ring Force/Point of Contact calc/z calc ==
  note: num = -(Zc - L/2 + r31*cos(th)*(rl + (Lcyl*(rl - rs))/(2*lc)) + r32*sin(th)*(rl + (Lcyl*(rl - rs))/(2*lc)))
      | den = (r33 + (r31*cos(th)*(rl - rs))/lc + (r32*sin(th)*(rl - rs))/lc)
  r31 : Inport
  r32 : Inport  Port=2
  r33 : Inport  Port=3
  zc : Inport  Port=4
  th : Inport  Port=5
  Constant : Constant  Value=(rl + (l_cyl*(rl - rs))/(2*lc))
  Constant1 : Constant  Value=l_tube/2
  Constant2 : Constant  Value=(rl - rs)/lc
  Divide : Product  Inputs=*/
  Gain : Gain  Gain=-1
  Product{,1..5} (6 alike) : Product
  Sum : Sum  Inputs=+-++
  Sum1 : Sum  Inputs=+++
  Trigonometric Function : Trigonometry  Operator=cos
  Trigonometric Function1 : Trigonometry
  z : Outport  VectorParamsAs1DForOutWhenUnconnected=off
  wires:
  Divide/1 -> z/1
  th/1 -> Trigonometric Function1/1, Trigonometric Function/1
  Trigonometric Function/1 -> Product/2
  r31/1 -> Product/1
  Trigonometric Function1/1 -> Product1/2
  r32/1 -> Product1/1
  zc/1 -> Sum/1
  Constant1/1 -> Sum/2
  Product2/1 -> Sum/3
  Product3/1 -> Sum/4
  Product/1 -> Product4/1, Product2/1
  Product1/1 -> Product3/1, Product5/1
  Constant/1 -> Product3/2, Product2/2
  Sum/1 -> Gain/1
  Product5/1 -> Sum1/3
  Product4/1 -> Sum1/2
  r33/1 -> Sum1/1
  Constant2/1 -> Product4/2, Product5/2
  Sum1/1 -> Divide/2
  Gain/1 -> Divide/1

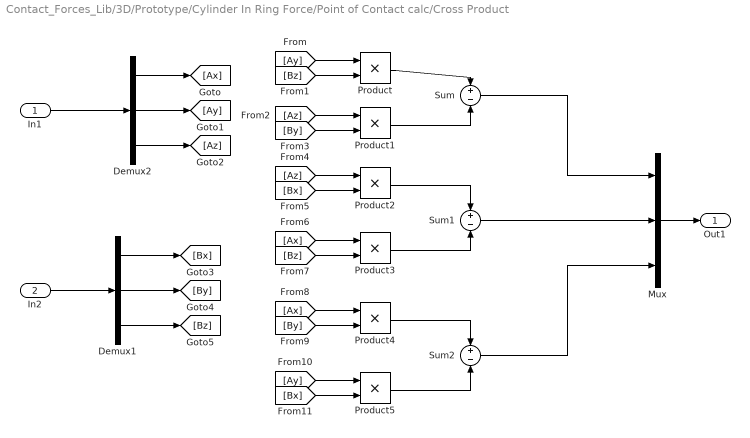
== system Contact_Forces_Lib/3D/Prototype/Cylinder In Ring Force/Point of Contact calc/Cross Product ==
  In1 : Inport
  In2 : Inport  Port=2
  Demux1 : Demux  Outputs=3
  Demux2 : Demux  Outputs=3
  Mux : Mux  Inputs=3
  Product{,1..5} (6 alike) : Product
  Sum : Sum  Inputs=+|-
  Sum1 : Sum  Inputs=+|-
  Sum2 : Sum  Inputs=+|-
  Out1 : Outport  VectorParamsAs1DForOutWhenUnconnected=off
  wires:
  [Bx] -> Product5/2
  [Ay] -> Product5/1
  [By] -> Product4/2
  [Ax] -> Product4/1
  [Bz] -> Product3/2
  [Ax] -> Product3/1
  [Bx] -> Product2/2
  [Az] -> Product2/1
  [By] -> Product1/2
  [Az] -> Product1/1
  [Bz] -> Product/2
  [Ay] -> Product/1
  Demux1/3 -> [Bz]
  Demux1/2 -> [By]
  Demux1/1 -> [Bx]
  Demux2/3 -> [Az]
  Demux2/2 -> [Ay]
  Demux2/1 -> [Ax]
  In1/1 -> Demux2/1
  Sum2/1 -> Mux/3
  Sum/1 -> Mux/1
  Sum1/1 -> Mux/2
  Product5/1 -> Sum2/2
  Product4/1 -> Sum2/1
  Product3/1 -> Sum1/2
  Product2/1 -> Sum1/1
  Product/1 -> Sum/1
  Product1/1 -> Sum/2
  Mux/1 -> Out1/1
  In2/1 -> Demux1/1

== system Contact_Forces_Lib/3D/Prototype/Cylinder In Ring Force/Point of Contact calc/Force Calc ==
  x : Inport
  y : Inport  Port=2
  v : Inport  Port=3
  z : Inport  Port=4
  th : Inport  Port=5
  Computing Force from nonzero penetration points : Subsystem  Commented=on
  Constant2 : Constant  Value=r_tube
  Dead Zone : DeadZone  LowerValue=-inf  UpperValue=0  ZeroCross=off
  MAX_ML : Subsystem  Commented=on
  MAX_SL : Subsystem
  Math Function : Math  Operator=square  SignedPower=on
  Math Function1 : Math  Operator=square  SignedPower=on
  Reciprocal Sqrt : Sqrt
  Sum : Sum  Inputs=|++
  Sum1 : Sum  Inputs=|+-
  Fx : Outport  VectorParamsAs1DForOutWhenUnconnected=off
  Fy : Outport  Port=2  VectorParamsAs1DForOutWhenUnconnected=off
  Fz : Outport  Port=3  VectorParamsAs1DForOutWhenUnconnected=off
  pc : Outport  Port=4  VectorParamsAs1DForOutWhenUnconnected=off
  maxpen : Outport  Port=5  VectorParamsAs1DForOutWhenUnconnected=off
  wires:
  y/1 -> MAX_SL/1(Y), Math Function1/1
  x/1 -> MAX_SL/2(X), Math Function/1
  Sum/1 -> Reciprocal Sqrt/1
  Reciprocal Sqrt/1 -> Sum1/1
  Constant2/1 -> Sum1/2
  Sum1/1 -> Dead Zone/1
  MAX_SL/1(Fx) -> Fx/1
  MAX_SL/2(Fy) -> Fy/1
  Dead Zone/1 -> MAX_SL/3(Pen)
  Math Function1/1 -> Sum/1
  Math Function/1 -> Sum/2
  v/1 -> MAX_SL/4(v)
  th/1 -> MAX_SL/5(th)
  z/1 -> MAX_SL/6(z)
  MAX_SL/4(pc) -> pc/1
  MAX_SL/3(Fz) -> Fz/1
  MAX_SL/5(maxpen) -> maxpen/1

== system Contact_Forces_Lib/3D/Prototype/Cylinder In Ring Force/Point of Contact calc/x calc ==
  note: Xb = r11*r*cos(th) + r12*r*sin(th) +r13*z + Xc;
  note: Find x coordinate in tube frame for cylinder point that is in the plane of the end of the tube
  r11 : Inport
  r12 : Inport  Port=2
  r13 : Inport  Port=3
  xc : Inport  Port=4
  th : Inport  Port=5
  z : Inport  Port=6
  Gain : Gain  Gain=r_cyl
  Gain1 : Gain  Gain=r_cyl
  Product : Product
  Product1 : Product
  Product2 : Product
  Sum : Sum  Inputs=|++++
  Trigonometric Function : Trigonometry  Operator=cos
  Trigonometric Function1 : Trigonometry
  x : Outport  VectorParamsAs1DForOutWhenUnconnected=off
  wires:
  th/1 -> Trigonometric Function/1, Trigonometric Function1/1
  Sum/1 -> x/1
  Product/1 -> Gain/1
  Gain1/1 -> Sum/3
  Trigonometric Function/1 -> Product/2
  Trigonometric Function1/1 -> Product1/2
  Gain/1 -> Sum/2
  Product1/1 -> Gain1/1
  r11/1 -> Product/1
  r12/1 -> Product1/1
  xc/1 -> Sum/1
  r13/1 -> Product2/1
  z/1 -> Product2/2
  Product2/1 -> Sum/4

== system Contact_Forces_Lib/3D/Prototype/Cylinder In Ring Force/Point of Contact calc/y calc ==
  note: Yb = r21*r*cos(th) + r22*r*sin(th) +r23*z + Yc;
  note: Find y coordinate in tube frame for cylinder point that is in the plane of the end of the tube
  r21 : Inport
  r22 : Inport  Port=2
  r23 : Inport  Port=3
  yc : Inport  Port=4
  th : Inport  Port=5
  z : Inport  Port=6
  Gain : Gain  Gain=r_cyl
  Gain1 : Gain  Gain=r_cyl
  Product : Product
  Product1 : Product
  Product2 : Product
  Sum : Sum  Inputs=|++++
  Trigonometric Function : Trigonometry  Operator=cos
  Trigonometric Function1 : Trigonometry
  y : Outport  VectorParamsAs1DForOutWhenUnconnected=off
  wires:
  Product2/1 -> Sum/4
  z/1 -> Product2/2
  r23/1 -> Product2/1
  yc/1 -> Sum/1
  r22/1 -> Product1/1
  r21/1 -> Product/1
  Product1/1 -> Gain1/1
  Gain/1 -> Sum/2
  Trigonometric Function1/1 -> Product1/2
  Trigonometric Function/1 -> Product/2
  Gain1/1 -> Sum/3
  Product/1 -> Gain/1
  Sum/1 -> y/1
  th/1 -> Trigonometric Function1/1, Trigonometric Function/1

== system Contact_Forces_Lib/3D/Prototype/Cylinder In Ring Force/Point of Contact calc/z calc ==
  note: Find z coordinate in cylinder frame for cylinder point that is in the plane of the end of the tube
  note: z = (L/2 - r31*r*cos(th) - r32*r*sin(th) - Zc)/r33;
  r31 : Inport
  r32 : Inport  Port=2
  r33 : Inport  Port=3
  zc : Inport  Port=4
  th : Inport  Port=5
  Constant : Constant  Value=l_tube/2
  Divide : Product  Inputs=*/
  Gain : Gain  Gain=r_cyl
  Gain1 : Gain  Gain=r_cyl
  Product : Product
  Product1 : Product
  Sum : Sum  Inputs=|---+
  Trigonometric Function : Trigonometry  Operator=cos
  Trigonometric Function1 : Trigonometry
  z : Outport  VectorParamsAs1DForOutWhenUnconnected=off
  wires:
  r32/1 -> Product1/1
  r31/1 -> Product/1
  Product1/1 -> Gain1/1
  Gain/1 -> Sum/2
  Trigonometric Function1/1 -> Product1/2
  Trigonometric Function/1 -> Product/2
  Gain1/1 -> Sum/3
  Product/1 -> Gain/1
  r33/1 -> Divide/2
  Constant/1 -> Sum/4
  Sum/1 -> Divide/1
  Divide/1 -> z/1
  zc/1 -> Sum/1
  th/1 -> Trigonometric Function1/1, Trigonometric Function/1

== system Contact_Forces_Lib/3D/Sphere in Sphere Force/Ff/Check w or v non zero/Else ==
  Action Port : ActionPort
  vabs_zero : Constant  Value=0  SampleTime=0
  vuvect_zero : Constant  Value=[0 0 0]  SampleTime=0
  vabs : Outport  InitialOutput=0  VectorParamsAs1DForOutWhenUnconnected=off
  vuvect : Outport  Port=2  InitialOutput=0  VectorParamsAs1DForOutWhenUnconnected=off
  wires:
  vabs_zero/1 -> vabs/1
  vuvect_zero/1 -> vuvect/1

== system Contact_Forces_Lib/3D/Sphere in Sphere Force/Ff/Check w or v non zero/mag v ==
  vect : Inport
  Add2 : Sum  Inputs=+++
  Demux : Demux  Outputs=3
  Math Function : Math  Operator=square  SignedPower=on
  Math Function1 : Math  Operator=square  SignedPower=on
  Math Function2 : Math  Operator=square  SignedPower=on
  Sqrt : Sqrt
  mag : Outport  VectorParamsAs1DForOutWhenUnconnected=off
  wires:
  Math Function2/1 -> Add2/3
  Demux/3 -> Math Function2/1
  Sqrt/1 -> mag/1
  Math Function1/1 -> Add2/2
  Math Function/1 -> Add2/1
  Add2/1 -> Sqrt/1
  vect/1 -> Demux/1
  Demux/1 -> Math Function/1
  Demux/2 -> Math Function1/1

== system Contact_Forces_Lib/3D/Sphere in Sphere Force/Ff/Check w or v non zero/mag w ==
  vect : Inport
  Add : Sum  Inputs=+++
  Demux : Demux  Outputs=3
  Math Function : Math  Operator=square  SignedPower=on
  Math Function1 : Math  Operator=square  SignedPower=on
  Math Function2 : Math  Operator=square  SignedPower=on
  Sqrt : Sqrt
  mag : Outport  VectorParamsAs1DForOutWhenUnconnected=off
  wires:
  Demux/2 -> Math Function1/1
  Demux/1 -> Math Function/1
  vect/1 -> Demux/1
  Add/1 -> Sqrt/1
  Math Function/1 -> Add/1
  Math Function1/1 -> Add/2
  Sqrt/1 -> mag/1
  Demux/3 -> Math Function2/1
  Math Function2/1 -> Add/3

== system Contact_Forces_Lib/3D/Sphere in Sphere Force/Ff/SlipVel/If Action Subsystem ==
  In1 : Inport
  In2 : Inport  Port=2
  Action Port : ActionPort
  Divide : Product  Inputs=/*
  Out1 : Outport  VectorParamsAs1DForOutWhenUnconnected=off
  wires:
  Divide/1 -> Out1/1
  In2/1 -> Divide/2
  In1/1 -> Divide/1

== system Contact_Forces_Lib/3D/Sphere in Sphere Force/Ff/SlipVel/mag ==
  vect : Inport
  Add2 : Sum  Inputs=+++
  Demux : Demux  Outputs=3
  Math Function : Math  Operator=square  SignedPower=on
  Math Function1 : Math  Operator=square  SignedPower=on
  Math Function2 : Math  Operator=square  SignedPower=on
  Sqrt : Sqrt
  mag : Outport  VectorParamsAs1DForOutWhenUnconnected=off
  wires:
  Math Function2/1 -> Add2/3
  Demux/3 -> Math Function2/1
  Sqrt/1 -> mag/1
  Math Function1/1 -> Add2/2
  Math Function/1 -> Add2/1
  Add2/1 -> Sqrt/1
  vect/1 -> Demux/1
  Demux/1 -> Math Function/1
  Demux/2 -> Math Function1/1

== system Contact_Forces_Lib/3D/Sphere to Cone Force/Forces/Ff/Relative vel at CP ==
  note: Calculate relative velocity at contact point between sphere and tube. Two components: about ring and along tube axis. Use magnitude to calculate friction force, atan2 retains relative magnitude and direction between the components.
  InOut : Inport
  rad : Inport  Port=2
  vrad : Inport  Port=3
  Pen : Inport  Port=4
  vazm : Inport  Port=5
  vazmx : Inport  Port=6
  vazmy : Inport  Port=7
  wzf : Inport  Port=8
  vzf : Inport  Port=9
  wxf : Inport  Port=10
  wyf : Inport  Port=11
  azm : Inport  Port=12
  Calculate vRelFace : Subsystem
  Calculate vRelRing : Subsystem
  Follower Radius : Constant  Value=radius_sphere
  Math Function : Math  Operator=square  SignedPower=on
  Math Function1 : Math  Operator=square  SignedPower=on
  Midpt Pen : Gain  Gain=0.5
  Product1 : Product
  Sqrt : Sqrt
  Sum1 : Sum  Inputs=+-
  Sum3 : Sum  Inputs=|++
  Trigonometric Function : Trigonometry  Operator=atan2
  vRelAbs : Outport  VectorParamsAs1DForOutWhenUnconnected=off
  rSphtoCP : Outport  Port=2  VectorParamsAs1DForOutWhenUnconnected=off
  rConAxtoCP : Outport  Port=3  VectorParamsAs1DForOutWhenUnconnected=off
  alpha : Outport  Port=4  VectorParamsAs1DForOutWhenUnconnected=off
  wires:
  vrad/1 -> Calculate vRelFace/6(vrad)
  vazmy/1 -> Calculate vRelRing/6(vazmy)
  vazmx/1 -> Calculate vRelRing/5(vazmx)
  Product1/1 -> Calculate vRelRing/1(rSphtoCP sign), Calculate vRelFace/1(rSphtoCP sign)
  Sum1/1 -> Product1/1, rSphtoCP/1  "rSphtoCP"
  InOut/1 -> Product1/2  "InOut"
  Trigonometric Function/1 -> alpha/1  "alpha"
  Sqrt/1 -> vRelAbs/1
  Sum3/1 -> Sqrt/1
  Math Function/1 -> Sum3/1
  Math Function1/1 -> Sum3/2
  Follower Radius/1 -> Sum1/1
  Pen/1 -> Midpt Pen/1
  Midpt Pen/1 -> Sum1/2
  Calculate vRelFace/1(vRelFace) -> Math Function1/1, Trigonometric Function/1  "vRelFace"
  wxf/1 -> Calculate vRelFace/3(wxf), Calculate vRelRing/8(wxf)
  vzf/1 -> Calculate vRelFace/5(vzf)
  azm/1 -> Calculate vRelFace/2(azm), Calculate vRelRing/7(azm)
  wyf/1 -> Calculate vRelRing/9(wyf), Calculate vRelFace/4(wyf)
  Calculate vRelRing/2(vRelRing) -> Math Function/1, Trigonometric Function/2  "vRelRing"
  rad/1 -> Calculate vRelRing/2(rad)
  vazm/1 -> Calculate vRelRing/3(vazm)
  wzf/1 -> Calculate vRelRing/4(wzf)
  Calculate vRelRing/1(rConAxtoCP) -> rConAxtoCP/1

== system Contact_Forces_Lib/3D/Sphere to Cone Force/Forces/Ff/Resolve Ff ==
  note: Resolve Friction Force in
      | Sphere F reference frame
  note: Resolve Friction Force in
      | Cone B reference frame
  InOut : Inport
  Ff : Inport  Port=2
  R : Inport  Port=3
  z : Inport  Port=4
  rSphtoCP : Inport  Port=5
  rConAxtoCP : Inport  Port=6
  alpha : Inport  Port=7
  azm : Inport  Port=8
  Ff in ConB : Subsystem
  Ff in SphF : Subsystem
  FxSphF : Outport  VectorParamsAs1DForOutWhenUnconnected=off
  FySphF : Outport  Port=2  VectorParamsAs1DForOutWhenUnconnected=off
  FzSphF : Outport  Port=3  VectorParamsAs1DForOutWhenUnconnected=off
  TSphF : Outport  Port=4  VectorParamsAs1DForOutWhenUnconnected=off
  FxConB : Outport  Port=5  VectorParamsAs1DForOutWhenUnconnected=off
  FyConB : Outport  Port=6  VectorParamsAs1DForOutWhenUnconnected=off
  FzConB : Outport  Port=7  VectorParamsAs1DForOutWhenUnconnected=off
  TConB : Outport  Port=8  VectorParamsAs1DForOutWhenUnconnected=off
  wires:
  Ff in SphF/4(TSphF) -> TSphF/1
  Ff in ConB/4(TSphF_B) -> Ff in SphF/4(TSphF_B)
  Ff in ConB/5(TConB) -> TConB/1
  alpha/1 -> Ff in ConB/4(alpha)
  Ff in ConB/3(FzConB) -> FzConB/1, Ff in SphF/3(FzConB)
  Ff in SphF/3(FzSphF) -> FzSphF/1
  R/1 -> Ff in SphF/5(R)
  azm/1 -> Ff in ConB/3(azm)
  Ff in SphF/2(FxSphF) -> FxSphF/1
  Ff in ConB/2(FyConB) -> Ff in SphF/2(FyConB), FyConB/1
  Ff in ConB/1(FxConB) -> FxConB/1, Ff in SphF/1(FxConB)
  Ff in SphF/1(FySphF) -> FySphF/1
  Ff/1 -> Ff in ConB/2(Ff)
  rConAxtoCP/1 -> Ff in ConB/6(rConAxtoCP)
  rSphtoCP/1 -> Ff in ConB/5(rSphtoCP)
  z/1 -> Ff in ConB/7(z)
  InOut/1 -> Ff in ConB/1(InOut)

== system Contact_Forces_Lib/3D/Sphere to Cone Force/Forces/Fn/Equiv Torques ==
  azm : Inport
  FxConB : Inport  Port=2
  FyConB : Inport  Port=3
  FzConB : Inport  Port=4
  rad : Inport  Port=5
  z : Inport  Port=6
  Constant : Constant  Value=radius_sphere*sinConeTh
  Constant1 : Constant  Value=radius_sphere*cosConeTh
  Product : Product  Inputs=3
  Product1 : Product
  Product2 : Product  Inputs=3
  Product3 : Product
  Sum : Sum
  Sum1 : Sum  Inputs=+-
  Sum2 : Sum
  Sum3 : Sum  Inputs=+-
  sin : Trigonometry
  sin1 : Trigonometry  Operator=cos
  TxConB : Outport  VectorParamsAs1DForOutWhenUnconnected=off
  TyConB : Outport  Port=2  VectorParamsAs1DForOutWhenUnconnected=off
  wires:
  sin1/1 -> Product2/2
  sin/1 -> Product/2
  Sum/1 -> Product/3, Product2/3
  Sum3/1 -> TyConB/1
  Sum1/1 -> TxConB/1
  rad/1 -> Sum/1
  Product3/1 -> Sum3/1
  Product/1 -> Sum1/1
  Constant1/1 -> Sum2/2
  Sum2/1 -> Product3/2, Product1/2
  Constant/1 -> Sum/2
  z/1 -> Sum2/1
  Product1/1 -> Sum1/2
  Product2/1 -> Sum3/2
  azm/1 -> sin/1, sin1/1
  FxConB/1 -> Product3/1
  FzConB/1 -> Product/1, Product2/1
  FyConB/1 -> Product1/1
